simulink subsystem "execute_command"  (R2026a)
settings: Solver=VariableStepAuto
undefined symbols (not defined in the file): S
PreSaveFcn:
  | defaultToFileBlockNames(bdroot);
settings Model: Creator=kjhaydon  LastModifiedBy=kjhaydon

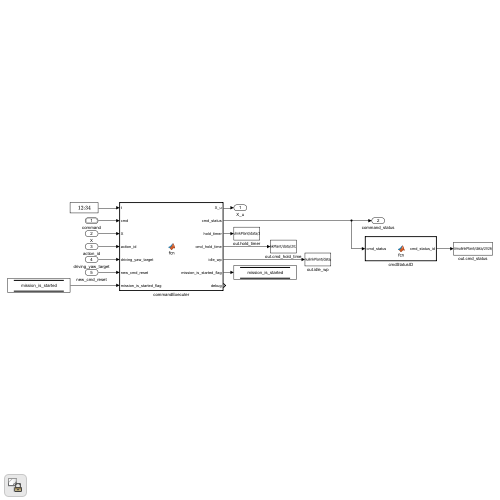
[thumbnail: Simulink's stored preview of the top-level diagram]
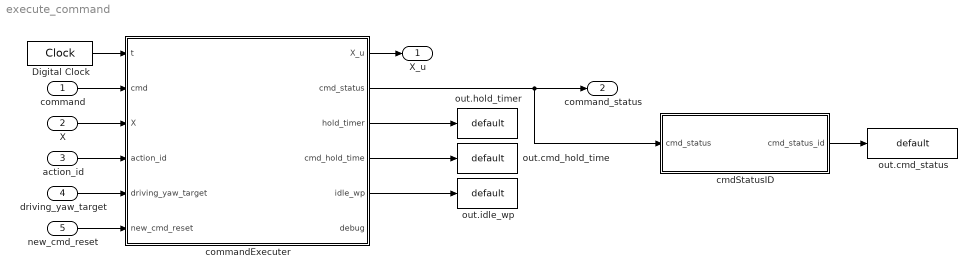
== system execute_command ==
  command : Inport  OutDataTypeStr=Bus: cmd_bus  SampleTime=S.dt_control
  X : Inport  Port=2  SampleTime=S.dt_control
  action_id : Inport  Port=3  SampleTime=S.dt_control
  driving_yaw_target : Inport  Port=4  SampleTime=S.dt_control
  new_cmd_reset : Inport  Port=5  SampleTime=S.dt_control
  Digital Clock : DigitalClock  SampleTime=S.dt_control
  cmdStatusID : MATLAB Function  TreatAsAtomicUnit=on
  commandExecuter : MATLAB Function  TreatAsAtomicUnit=on
  out.cmd_hold_time : ToFile  Filename=default  MatrixName=cmd_hold_time  SaveFormat=Timeseries
  out.cmd_status : ToFile  Filename=default  MatrixName=cmd_status  SaveFormat=Timeseries
  out.hold_timer : ToFile  Filename=default  MatrixName=hold_timer  SaveFormat=Timeseries
  out.idle_wp : ToFile  Filename=default  MatrixName=idle_wp  SaveFormat=Timeseries
  X_u : Outport
  command_status : Outport  Port=2
  wires:
  commandExecuter/1(X_u) -> X_u/1
  commandExecuter/2(cmd_status) -> cmdStatusID/1(cmd_status), command_status/1
  cmdStatusID/1(cmd_status_id) -> out.cmd_status/1
  commandExecuter/3(hold_timer) -> out.hold_timer/1
  commandExecuter/4(cmd_hold_time) -> out.cmd_hold_time/1
  commandExecuter/5(idle_wp) -> out.idle_wp/1
  new_cmd_reset/1 -> commandExecuter/6(new_cmd_reset)
  action_id/1 -> commandExecuter/4(action_id)
  driving_yaw_target/1 -> commandExecuter/5(driving_yaw_target)
  command/1 -> commandExecuter/2(cmd)
  X/1 -> commandExecuter/3(X)
  Digital Clock/1 -> commandExecuter/1(t)

== matlab function execute_command/cmdStatusID ==
  settings: updateMethod=DISCRETE  sampleTime=S.dt_control
  data: cmd_status_id output; cmd_status input
function cmd_status_id = fcn(cmd_status)

cmd_status_id = cmdStatusID(cmd_status);

== matlab function execute_command/commandExecuter ==
  settings: updateMethod=DISCRETE  sampleTime=S.dt_control
  data: X_u output Bus: X_bus; cmd_status output int8 size=[4 1]; hold_timer output; cmd_hold_time output; idle_wp output; t input; cmd input; X input; action_id input; driving_yaw_target input; new_cmd_reset input; debug output
function [X_u, cmd_status, hold_timer, cmd_hold_time, idle_wp, debug]  = fcn(t, cmd, X, action_id, driving_yaw_target,new_cmd_reset)

[X_u, cmd_status, hold_timer, cmd_hold_time, idle_wp,debug] = commandExecuter(t, cmd, X, action_id, driving_yaw_target,new_cmd_reset);
